simulink model "im_inv_sensorless_ctrl_model"  (R2026a)
settings: Solver=ode1  StopTime=simlength  FixedStep=tc  MaxStep=tc  EnableMultiTasking=on
values from neighbouring files (symbols this model uses):
  cp = 2    [im_param_calc_3.m]
  Ibez = Inom*sqrt(2)    [im_param_calc_3.m]
  Lm = Ls - Lds    [im_param_calc_3.m]
  Lr = Lm + Ldr    [im_param_calc_3.m]
  Ls = Vnom/sqrt(3)/I0/(2*pi*fnom)    [im_param_calc_3.m]
  Rr = Rr+deltaRr    (= 0.00099)    [im_param_calc_3.m]
  Rs = PhaseResistance    (= 0.009)    [im_param_calc_3.m]
undefined symbols (not defined in the file or in its folder): Adrso_im, alpha_norm, beta_norm, Crso_im, CTRPIFF_CLIP_RELEASE, dead_time, DiscIntNeverNeededParam, emf_fb_p, emf_p, fi_rot_ref_norm, fPWM_INV, gamma_norm, iq_lim, Jm_model, kg, ki_inv_d, ki_inv_q, ki_w, kp_inv_d, kp_inv_q, kp_w, kw, Ldrso_im, Lm_norm, Lr_norm, Ls_norm, magnitude, Omega_r_bez, Omega_s_bez, Rs_norm, sigma_norm, simlength, tc, Tcontrol_INV, timeRamp, Tload, ts_afe, ts_inv, uf_omega_ref, uf_uq_ref, wref
libraries: nesl_utility x64, fl_lib x49, simulink x2, im_uvw_2_lib x1, threephase_inductor_lib x1, cstblocks_lti x1
(part 1 of 4)
settings Model: SimulationMode=accelerator  Creator=LTNBDA  LastModifiedBy=ltnbda
settings SolverCC: ZeroCrossControl=EnableAll
settings DataIOCC: MaxDataPoints=1  SignalLoggingSaveFormat=ModelDataLogs
settings OptimizationCC: InitFltsAndDblsToZero=on
settings DebuggingCC: SaveWithParameterizedLinksMsg=none  UnderspecifiedInitializationDetection=Classic  SignalResolutionControl=TryResolveAllWithWarning  MultiTaskDSMMsg=warning  MultiTaskCondExecSysMsg=none  MultiTaskRateTransMsg=warning
settings HardwareCC: ProdBitPerLong=64.0  ProdHWDeviceType=Generic->64-bit Embedded Processor (LP64)
settings SFSimCC: SimCustomHeaderCode=|
  | #include "mavgflt.h"
  | #include "mavgflt_simulink.h"
  | #include "bemf_obsv.h"
  | #include "bemf_obsv_simulink.h"
  | #include "bemf_obsv_load_est.h"
  | #include "bemf_obsv_load_est_simulink.h"
  | #include "dqvector_pi.h"
  | #include "dqvector_pi_simulink.h"
  | #include "sv_pwm_simulink.h"
  | #include "sv_pwm.h"
settings SFSimCC: SimUserSources=|
  | "mavgflt_simulink.c"
  | "mavgflt.c"
  | "bemf_obsv_simulink.c"
  | "bemf_obsv.c"
  | "bemf_obsv_load_est_simulink.c"
  | "bemf_obsv_load_est.c"
  | "dqvector_pi.c"
  | "dqvector_pi_simulink.c"
  | "sv_pwm_simulink.c"
  | "sv_pwm.c"
settings SFSimCC: SimUserIncludeDirs=|
  | include
  | src
settings GRTTargetCC: TargetFcnLib=ansi_tfl_tmw.mat  CombineOutputUpdateFcns=off  GRTInterface=on
settings SimscapeCC: SimscapeNormalizeSystem=off  SimscapeNominalValues="[{\"value\":\"1\",\"unit\":\"A\"},{\"value\":\"1\",\"unit\":\"bar\"},{\"value\":\"1\",\"unit\":\"cm^2\"},{\"value\":\"1\",\"unit\":\"cm^3/s\"},{\"value\":\"1\",\"unit\":\"kJ/kg\"},{\"value\":\"1\",\"unit\":\"kW\"},{\"value\":\"1\",\"unit\":\"l\"},{\"value\":\"1\",\"unit\":\"N\"},{\"value\":\"1\",\"unit\":\"N*m\"},{\"value\":\"1\",\"unit\":\"V\"}]"  SimscapeLogType=none  SimscapeLogDataHistory=5000.0

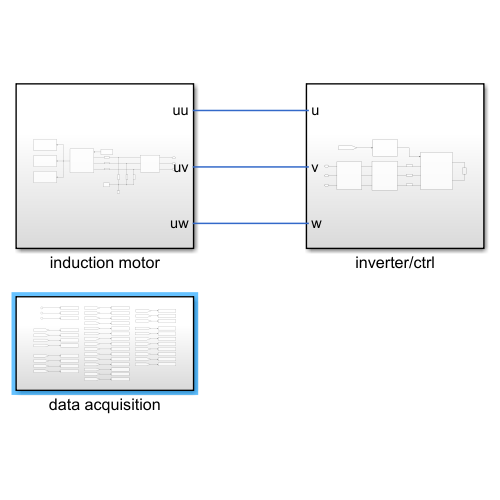
[thumbnail: Simulink's stored preview of the top-level diagram]
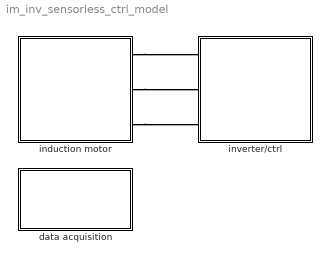
== system im_inv_sensorless_ctrl_model ==
  data acquisition : Subsystem
  induction motor : Subsystem
  inverter/ctrl : Subsystem
  connections:
  induction motor/RConn1 -- inverter/ctrl/LConn1
  induction motor/RConn2 -- inverter/ctrl/LConn2
  induction motor/RConn3 -- inverter/ctrl/LConn3

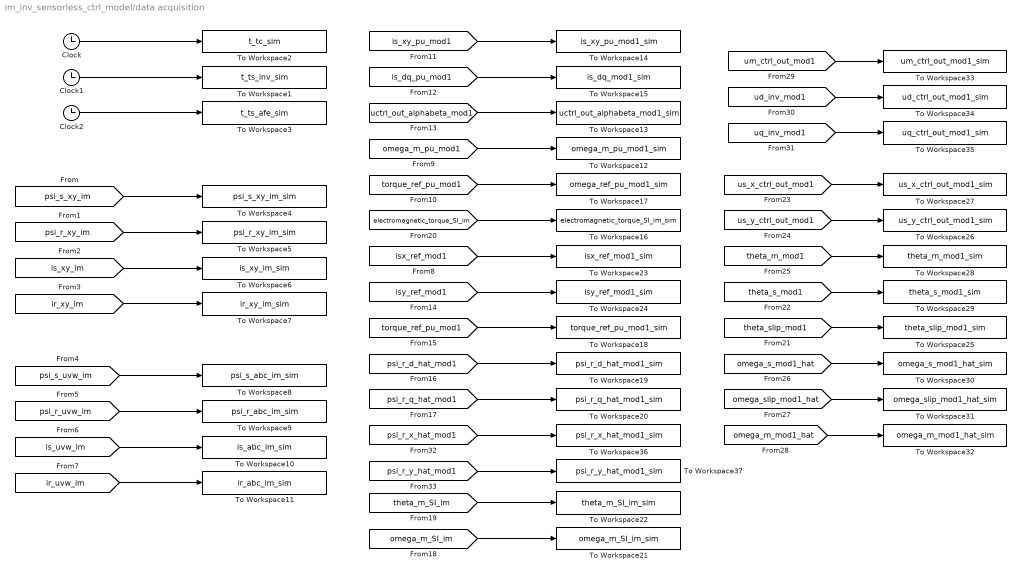
== system im_inv_sensorless_ctrl_model/data acquisition ==
  Clock : Clock
  Clock1 : Clock
  Clock2 : Clock
  To Workspace1 : ToWorkspace  VariableName=t_ts_inv_sim  SampleTime=ts_inv
      settings: MaxDataPoints=Ns_inv
  To Workspace10 : ToWorkspace  VariableName=is_abc_im_sim  SampleTime=tc
      settings: MaxDataPoints=Nc
  To Workspace11 : ToWorkspace  VariableName=ir_abc_im_sim  SampleTime=tc
      settings: MaxDataPoints=Nc
  To Workspace12 : ToWorkspace  VariableName=omega_m_pu_mod1_sim  SampleTime=ts_inv
      settings: MaxDataPoints=Ns_inv
  To Workspace13 : ToWorkspace  VariableName=uctrl_out_alphabeta_mod1_sim  SampleTime=ts_inv
      settings: MaxDataPoints=Ns_inv
  To Workspace14 : ToWorkspace  VariableName=is_xy_pu_mod1_sim  SampleTime=ts_inv
      settings: MaxDataPoints=Ns_inv
  To Workspace15 : ToWorkspace  VariableName=is_dq_mod1_sim  SampleTime=ts_inv
      settings: MaxDataPoints=Ns_inv
  To Workspace16 : ToWorkspace  VariableName=electromagnetic_torque_SI_im_sim  SampleTime=ts_inv
      settings: MaxDataPoints=Ns_inv
  To Workspace17 : ToWorkspace  VariableName=omega_ref_pu_mod1_sim  SampleTime=ts_inv
      settings: MaxDataPoints=Ns_inv
  To Workspace18 : ToWorkspace  VariableName=torque_ref_pu_mod1_sim  SampleTime=ts_inv
      settings: MaxDataPoints=Ns_inv
  To Workspace19 : ToWorkspace  VariableName=psi_r_d_hat_mod1_sim  SampleTime=ts_inv
      settings: MaxDataPoints=Ns_inv
  To Workspace2 : ToWorkspace  VariableName=t_tc_sim  SampleTime=tc
      settings: MaxDataPoints=Nc
  To Workspace20 : ToWorkspace  VariableName=psi_r_q_hat_mod1_sim  SampleTime=ts_inv
      settings: MaxDataPoints=Ns_inv
  To Workspace21 : ToWorkspace  VariableName=omega_m_SI_im_sim  SampleTime=ts_inv
      settings: MaxDataPoints=Ns_inv
  To Workspace22 : ToWorkspace  VariableName=theta_m_SI_im_sim  SampleTime=ts_inv
      settings: MaxDataPoints=Ns_inv
  To Workspace23 : ToWorkspace  VariableName=isx_ref_mod1_sim  SampleTime=ts_inv
      settings: MaxDataPoints=Ns_inv
  To Workspace24 : ToWorkspace  VariableName=isy_ref_mod1_sim  SampleTime=ts_inv
      settings: MaxDataPoints=Ns_inv
  To Workspace25 : ToWorkspace  VariableName=theta_slip_mod1_sim  SampleTime=ts_inv
      settings: MaxDataPoints=Ns_inv
  To Workspace26 : ToWorkspace  VariableName=us_y_ctrl_out_mod1_sim  SampleTime=ts_inv
      settings: MaxDataPoints=Ns_afe
  To Workspace27 : ToWorkspace  VariableName=us_x_ctrl_out_mod1_sim  SampleTime=ts_inv
      settings: MaxDataPoints=Ns_afe
  To Workspace28 : ToWorkspace  VariableName=theta_m_mod1_sim  SampleTime=ts_inv
      settings: MaxDataPoints=Ns_inv
  To Workspace29 : ToWorkspace  VariableName=theta_s_mod1_sim  SampleTime=ts_inv
      settings: MaxDataPoints=Ns_inv
  To Workspace3 : ToWorkspace  VariableName=t_ts_afe_sim  SampleTime=ts_afe
      settings: MaxDataPoints=Ns_afe
  To Workspace30 : ToWorkspace  VariableName=omega_s_mod1_hat_sim  SampleTime=ts_inv
      settings: MaxDataPoints=Ns_inv
  To Workspace31 : ToWorkspace  VariableName=omega_slip_mod1_hat_sim  SampleTime=ts_inv
      settings: MaxDataPoints=Ns_inv
  To Workspace32 : ToWorkspace  VariableName=omega_m_mod1_hat_sim  SampleTime=ts_inv
      settings: MaxDataPoints=Ns_inv
  To Workspace33 : ToWorkspace  VariableName=um_ctrl_out_mod1_sim  SampleTime=ts_inv
      settings: MaxDataPoints=Ns_afe
  To Workspace34 : ToWorkspace  VariableName=ud_ctrl_out_mod1_sim  SampleTime=ts_inv
      settings: MaxDataPoints=Ns_afe
  To Workspace35 : ToWorkspace  VariableName=uq_ctrl_out_mod1_sim  SampleTime=ts_inv
      settings: MaxDataPoints=Ns_afe
  To Workspace36 : ToWorkspace  VariableName=psi_r_x_hat_mod1_sim  SampleTime=ts_inv
      settings: MaxDataPoints=Ns_inv
  To Workspace37 : ToWorkspace  VariableName=psi_r_y_hat_mod1_sim  SampleTime=ts_inv
      settings: MaxDataPoints=Ns_inv
  To Workspace4 : ToWorkspace  VariableName=psi_s_xy_im_sim  SampleTime=tc
      settings: MaxDataPoints=Nc
  To Workspace5 : ToWorkspace  VariableName=psi_r_xy_im_sim  SampleTime=tc
      settings: MaxDataPoints=Nc
  To Workspace6 : ToWorkspace  VariableName=is_xy_im_sim  SampleTime=tc
      settings: MaxDataPoints=Nc
  To Workspace7 : ToWorkspace  VariableName=ir_xy_im_sim  SampleTime=tc
      settings: MaxDataPoints=Nc
  To Workspace8 : ToWorkspace  VariableName=psi_s_abc_im_sim  SampleTime=tc
      settings: MaxDataPoints=Nc
  To Workspace9 : ToWorkspace  VariableName=psi_r_abc_im_sim  SampleTime=tc
      settings: MaxDataPoints=Nc
  wires:
  Clock/1 -> To Workspace2/1
  Clock1/1 -> To Workspace1/1
  Clock2/1 -> To Workspace3/1
  [psi_s_xy_im] -> To Workspace4/1
  [psi_r_xy_im] -> To Workspace5/1
  [is_xy_im] -> To Workspace6/1
  [ir_xy_im] -> To Workspace7/1
  [psi_s_uvw_im] -> To Workspace8/1
  [psi_r_uvw_im] -> To Workspace9/1
  [is_uvw_im] -> To Workspace10/1
  [ir_uvw_im] -> To Workspace11/1
  [is_dq_pu_mod1] -> To Workspace15/1
  [uctrl_out_alphabeta_mod1] -> To Workspace13/1
  [is_xy_pu_mod1] -> To Workspace14/1
  [omega_m_pu_mod1] -> To Workspace12/1
  [electromagnetic_torque_SI_im] -> To Workspace16/1
  [torque_ref_pu_mod1] -> To Workspace17/1
  [omega_m_SI_im] -> To Workspace21/1
  [torque_ref_pu_mod1] -> To Workspace18/1
  [psi_r_d_hat_mod1] -> To Workspace19/1
  [psi_r_q_hat_mod1] -> To Workspace20/1
  [theta_m_SI_im] -> To Workspace22/1
  [isx_ref_mod1] -> To Workspace23/1
  [isy_ref_mod1] -> To Workspace24/1
  [theta_slip_mod1] -> To Workspace25/1
  [us_x_ctrl_out_mod1] -> To Workspace27/1
  [us_y_ctrl_out_mod1] -> To Workspace26/1
  [theta_m_mod1] -> To Workspace28/1
  [theta_s_mod1] -> To Workspace29/1
  [omega_s_mod1_hat] -> To Workspace30/1
  [omega_slip_mod1_hat] -> To Workspace31/1
  [omega_m_mod1_hat] -> To Workspace32/1
  [um_ctrl_out_mod1] -> To Workspace33/1
  [ud_inv_mod1] -> To Workspace34/1
  [uq_inv_mod1] -> To Workspace35/1
  [psi_r_x_hat_mod1] -> To Workspace36/1
  [psi_r_y_hat_mod1] -> To Workspace37/1

== system im_inv_sensorless_ctrl_model/induction motor ==
  Electrical Reference : fl_lib/Electrical/Electrical Elements/Electrical Reference
  Inductor : fl_lib/Electrical/Electrical Elements/Inductor  l=1e-6 H  r=0 Ohm  g=1e-9 1/Ohm  i_specify=off  i_priority=None  i=0 A  i_nominal_specify=off  i_nominal_value=1  i_nominal_unit=A  v_specify=off  v_priority=None  v=0 V  v_nominal_specify=off  v_nominal_value=1  v_nominal_unit=V  i_L_specify=off  i_L_priority=High  i_L=0 A  i_L_nominal_specify=off  i_L_nominal_value=1  i_L_nominal_unit=A
  Inductor1 : fl_lib/Electrical/Electrical Elements/Inductor  l=1e-6 H  r=0 Ohm  g=1e-9 1/Ohm  i_specify=off  i_priority=None  i=0 A  i_nominal_specify=off  i_nominal_value=1  i_nominal_unit=A  v_specify=off  v_priority=None  v=0 V  v_nominal_specify=off  v_nominal_value=1  v_nominal_unit=V  i_L_specify=off  i_L_priority=High  i_L=0 A  i_L_nominal_specify=off  i_L_nominal_value=1  i_L_nominal_unit=A
  Inductor2 : fl_lib/Electrical/Electrical Elements/Inductor  l=1e-6 H  r=0 Ohm  g=1e-9 1/Ohm  i_specify=off  i_priority=None  i=0 A  i_nominal_specify=off  i_nominal_value=1  i_nominal_unit=A  v_specify=off  v_priority=None  v=0 V  v_nominal_specify=off  v_nominal_value=1  v_nominal_unit=V  i_L_specify=off  i_L_priority=High  i_L=0 A  i_L_nominal_specify=off  i_L_nominal_value=1  i_L_nominal_unit=A
  Resistor : fl_lib/Electrical/Electrical Elements/Resistor  R=1e5 Ohm  i_specify=off  i_priority=None  i=0 A  i_nominal_specify=off  i_nominal_value=1  i_nominal_unit=A  v_specify=off  v_priority=None  v=0 V  v_nominal_specify=off  v_nominal_value=1  v_nominal_unit=V
  Resistor1 : fl_lib/Electrical/Electrical Elements/Resistor  R=1e5 Ohm  i_specify=off  i_priority=None  i=0 A  i_nominal_specify=off  i_nominal_value=1  i_nominal_unit=A  v_specify=off  v_priority=None  v=0 V  v_nominal_specify=off  v_nominal_value=1  v_nominal_unit=V
  Resistor2 : fl_lib/Electrical/Electrical Elements/Resistor  R=1e5 Ohm  i_specify=off  i_priority=None  i=0 A  i_nominal_specify=off  i_nominal_value=1  i_nominal_unit=A  v_specify=off  v_priority=None  v=0 V  v_nominal_specify=off  v_nominal_value=1  v_nominal_unit=V
  Solver Configuration : nesl_utility/Solver Configuration  PhysicalDomain=network_engine_domain  SubClassName=solver  LeftPortType=input  RightPortType=generic  Tones=[]  Harmonics=[]  SimulateNoise=off  Profile=off  UseLocalSampling=off  EnableSwitchedLinearOptims=on  FrequencyDomain=off  UseCCode=off  RelTol=0.001  AbsTol=0.001  MinStep=1e-09  ToWorkspace=off  RevertToSquareIcSolve=off  NumHomotopyIterations=100  PhasorMode=off  PhasorModeNumHarmonics=1  ConsistencySolver=NEWTON_XTOL_AFTER_FTOL  CanonicalOrdering=UNORDERED  OptimizeIntermediates=UNOPTIMIZED  IndexReductionMethod=DerivativeReplacement  DoDC=off  ResidualTolerance=1e-09  ConsistencyTolSource=GLOBAL  ConsistencyAbsTol=0.001  ConsistencyRelTol=0.001  ConsistencyTolFactor=0.001  UseLocalSolver=on  LocalSolverChoice=NE_BACKWARD_EULER_ADVANCER  ResolveIndetEquations=on  FunctionEvalNumThread=1  LocalSolverSampleTime=tc  DoFixedCost=on  MaxNonlinIter=3  MaxModeIter=2  ComputeImpulses=off  ImpulseIterations=2  LinearAlgebra=auto  LinearAlgebraNumThread=0  EquationFormulation=NE_TIME_EF  DelaysMemoryBudget=1024  AutomaticFiltering=on  FilteringTimeConstant=0.001  PartitionStorageMethod=AS_NEEDED  PartitionMemoryBudget=1024  PartitionMethod=ROBUST  MultibodyUseLocalSolver=off  MultibodyLocalSolverChoice=ODE1  MultibodyLocalSolverSampleTime=0.001
  control performance evaluation : Subsystem
  induction motor : Subsystem
  load generator : Subsystem
  machine performance evaluation : Subsystem
  mechanical data : Subsystem
  threephase_vi_measures_stack : Subsystem
  uu : PMIOPort  Side=Right
  uv : PMIOPort  Port=2  Side=Right
  uw : PMIOPort  Port=3  Side=Right
  wires:
  induction motor/1(motor_data) -> control performance evaluation/1(machine_data), machine performance evaluation/1(machine_data), mechanical data/1(machine data)
  load generator/1(torque) -> induction motor/1(torque load)
  connections:
  induction motor/LConn2 -- Inductor1/LConn1
  Resistor/LConn1 -- threephase_vi_measures_stack/RConn1 -- Inductor/RConn1
  induction motor/LConn3 -- Inductor2/LConn1
  induction motor/LConn1 -- Inductor/LConn1
  Resistor1/LConn1 -- threephase_vi_measures_stack/RConn2 -- Inductor1/RConn1
  Resistor2/LConn1 -- threephase_vi_measures_stack/RConn3 -- Inductor2/RConn1
  Resistor/RConn1 -- Solver Configuration/RConn1 -- Resistor2/RConn1 -- Resistor1/RConn1 -- Electrical Reference/LConn1
  threephase_vi_measures_stack/LConn1 -- uu/RConn1
  threephase_vi_measures_stack/LConn2 -- uv/RConn1
  threephase_vi_measures_stack/LConn3 -- uw/RConn1

== system im_inv_sensorless_ctrl_model/inverter//ctrl ==
  DC Voltage Source : fl_lib/Electrical/Electrical Sources/DC Voltage Source  v0=Vdc_ref V
  Inductor : fl_lib/Electrical/Electrical Elements/Inductor  l=1e-6 H  r=0 Ohm  g=1e-9 1/Ohm  i_specify=off  i_priority=None  i=0 A  i_nominal_specify=off  i_nominal_value=1  i_nominal_unit=A  v_specify=off  v_priority=None  v=0 V  v_nominal_specify=off  v_nominal_value=1  v_nominal_unit=V  i_L_specify=off  i_L_priority=High  i_L=0 A  i_L_nominal_specify=off  i_L_nominal_value=1  i_L_nominal_unit=A
  Inductor1 : fl_lib/Electrical/Electrical Elements/Inductor  l=1e-6 H  r=0 Ohm  g=1e-9 1/Ohm  i_specify=off  i_priority=None  i=0 A  i_nominal_specify=off  i_nominal_value=1  i_nominal_unit=A  v_specify=off  v_priority=None  v=0 V  v_nominal_specify=off  v_nominal_value=1  v_nominal_unit=V  i_L_specify=off  i_L_priority=High  i_L=0 A  i_L_nominal_specify=off  i_L_nominal_value=1  i_L_nominal_unit=A
  Inductor2 : fl_lib/Electrical/Electrical Elements/Inductor  l=1e-6 H  r=0 Ohm  g=1e-9 1/Ohm  i_specify=off  i_priority=None  i=0 A  i_nominal_specify=off  i_nominal_value=1  i_nominal_unit=A  v_specify=off  v_priority=None  v=0 V  v_nominal_specify=off  v_nominal_value=1  v_nominal_unit=V  i_L_specify=off  i_L_priority=High  i_L=0 A  i_L_nominal_specify=off  i_L_nominal_value=1  i_L_nominal_unit=A
  LFi : threephase_inductor_lib/threephase inductor  Lp=LFi_d H  L0=LFi_0 H  Rp=RLFi_d Ohm  R0=RLFi_0 Ohm  Lls=5e-6 H  uu_1_specify=off  uu_1_priority=None  uu_1=0 V  uu_1_nominal_specify=off  uu_1_nominal_value=1  uu_1_nominal_unit=V  uv_1_specify=off  uv_1_priority=None  uv_1=0 V  uv_1_nominal_specify=off  uv_1_nominal_value=1  uv_1_nominal_unit=V  uw_1_specify=off  uw_1_priority=None  uw_1=0 V  uw_1_nominal_specify=off  uw_1_nominal_value=1  uw_1_nominal_unit=V  uu_2_specify=off  uu_2_priority=None  uu_2=0 V  uu_2_nominal_specify=off  uu_2_nominal_value=1  uu_2_nominal_unit=V  uv_2_specify=off  uv_2_priority=None  uv_2=0 V  uv_2_nominal_specify=off  uv_2_nominal_value=1  uv_2_nominal_unit=V  uw_2_specify=off  uw_2_priority=None  uw_2=0 V  uw_2_nominal_specify=off  uw_2_nominal_value=1  uw_2_nominal_unit=V  iu_specify=off  iu_priority=None  iu=0 A  iu_nominal_specify=off  iu_nominal_value=1  iu_nominal_unit=A  iv_specify=off  iv_priority=None  iv=0 A  iv_nominal_specify=off  iv_nominal_value=1  iv_nominal_unit=A  iw_specify=off  iw_priority=None  iw=0 A  iw_nominal_specify=off  iw_nominal_value=1  iw_nominal_unit=A
  im_ctrl : Subsystem
  inverter : Subsystem
  threephase_vi_measures_stack : Subsystem
  u : PMIOPort  Side=Left
  v : PMIOPort  Port=2  Side=Left
  w : PMIOPort  Port=3  Side=Left
  wires:
  [theta_m_mod1] -> im_ctrl/1(theta_m)
  im_ctrl/1(u_ctrl_alphabeta) -> inverter/1(uab)
  connections:
  LFi/RConn1 -- Inductor/LConn1
  Inductor1/LConn1 -- LFi/RConn2
  LFi/RConn3 -- Inductor2/LConn1
  threephase_vi_measures_stack/LConn1 -- LFi/LConn1
  threephase_vi_measures_stack/LConn2 -- LFi/LConn2
  threephase_vi_measures_stack/LConn3 -- LFi/LConn3
  threephase_vi_measures_stack/RConn3 -- w/RConn1
  threephase_vi_measures_stack/RConn2 -- v/RConn1
  threephase_vi_measures_stack/RConn1 -- u/RConn1
  inverter/LConn1 -- Inductor/RConn1
  inverter/LConn2 -- Inductor1/RConn1
  inverter/LConn3 -- Inductor2/RConn1
  DC Voltage Source/LConn1 -- inverter/RConn1
  DC Voltage Source/RConn1 -- inverter/RConn2

== system im_inv_sensorless_ctrl_model/induction motor/control performance evaluation ==
  machine_data : Inport
  adc2dq_s_1 : Subsystem
  adc2dq_s_2 : Subsystem
  adc2dq_slip_1 : Subsystem
  adc2dq_slip_2 : Subsystem
  ir_uvw : BusSelector  OutputSignals=iru(A),irv(A),irw(A)  OutputAsBus=on
  is_uvw : BusSelector  OutputSignals=isu(A),isv(A),isw(A)  OutputAsBus=on
  psi_r_uvw : BusSelector  OutputSignals=psi_r_u(Vs),psi_r_v(Vs),psi_r_w(Vs)  OutputAsBus=on
  psi_s_uvw : BusSelector  OutputSignals=psi_s_u(Vs),psi_s_v(Vs),psi_s_w(Vs)  OutputAsBus=on
  stator/rotor uvw currents : Scope  NumInputPorts=2
      settings: ActiveDisplayYMinimum=-569.7187250347755  ActiveDisplayYMaximum=580.7473381124961  DataLoggingVariableName=ScopeData15
  stator/rotor uvw fluxes : Scope  NumInputPorts=2
      settings: ActiveDisplayYMinimum=-1.236467692960036  ActiveDisplayYMaximum=1.3517472693614645  DataLoggingVariableName=ScopeData16
  stator/rotor xy currents : Scope  NumInputPorts=2
      settings: ActiveDisplayYMinimum=-2297.8110392737149  ActiveDisplayYMaximum=257.87338844640192
  stator/rotor xy fluxes : Scope  NumInputPorts=2
      settings: ActiveDisplayYMinimum=-2.073456127351001  ActiveDisplayYMaximum=0.70751576648044434  DataLoggingVariableName=ScopeData2
  tag scope: ir_uvw_im=global, is_uvw_im=global, psi_r_uvw_im=global, psi_s_uvw_im=global
  wires:
  machine_data/1 -> psi_s_uvw/1, psi_r_uvw/1, is_uvw/1, ir_uvw/1
  psi_s_uvw/1 -> [psi_s_uvw_im], adc2dq_s_1/1(abc)
  adc2dq_s_1/1(dq) -> stator/rotor xy fluxes/1  "psi_s_xy"
  psi_r_uvw/1 -> [psi_r_uvw_im], adc2dq_slip_1/1(abc)
  adc2dq_slip_1/1(dq) -> stator/rotor xy fluxes/2  "psi_r_xy"
  adc2dq_slip_2/1(dq) -> stator/rotor xy currents/2  "ir_xy"
  adc2dq_s_2/1(dq) -> stator/rotor xy currents/1  "is_xy"
  is_uvw/1 -> [is_uvw_im], adc2dq_s_2/1(abc)
  ir_uvw/1 -> [ir_uvw_im], adc2dq_slip_2/1(abc)
  [is_uvw_im] -> stator/rotor uvw currents/1
  [ir_uvw_im] -> stator/rotor uvw currents/2
  [psi_r_uvw_im] -> stator/rotor uvw fluxes/2
  [psi_s_uvw_im] -> stator/rotor uvw fluxes/1

== system im_inv_sensorless_ctrl_model/induction motor/induction motor ==
  torque load : Inport
  Gain : Gain  Gain=-1
  Ideal Rotational Motion Sensor : fl_lib/Mechanical/Mechanical Sensors/Ideal Rotational Motion Sensor  reference=foundation.enum.MeasurementReference.difference  acceleration_port=false  velocity_port=true  position_port=true  wrap_angle=false  offset=0 rad
  Ideal Torque Source : fl_lib/Mechanical/Mechanical Sources/Ideal Torque Source
  Mechanical Rotational Reference : fl_lib/Mechanical/Rotational Elements/Mechanical Rotational Reference
  Mechanical Rotational Reference1 : fl_lib/Mechanical/Rotational Elements/Mechanical Rotational Reference
  Open Circuit : fl_lib/Electrical/Electrical Elements/Open Circuit  v_specify=off  v_priority=None  v=0 V  v_nominal_specify=off  v_nominal_value=1  v_nominal_unit=V
  PS Gain : fl_lib/Physical Signals/Functions/PS Gain  gain=-1
  PS Transfer Function : fl_lib/Physical Signals/Linear Operators/PS Transfer Function  transfer_function_type=foundation.enum.transfer_function_type.lag  T=1/50 s  T1=2 s  T2=1 s  reset_method=foundation.enum.IntegratorResetSpec.None  initial_condition_spec=foundation.enum.IntegratorICSpec.Internal  y0=0 N*m
  PS-Simulink Converter24 : nesl_utility/PS-Simulink Converter  PhysicalDomain=network_engine_domain  SubClassName=ps_output  LeftPortType=input  RightPortType=output  PseudoPeriodic=off  Frequencies=[]  VectorFormat=1-D array  Unit=rad  AffineConversion=off
  Simulink-PS Converter : nesl_utility/Simulink-PS Converter  PhysicalDomain=network_engine_domain  SubClassName=ps_input  LeftPortType=input  RightPortType=output  PseudoPeriodic=off  Frequencies=[]  NoiseDistribution=none  NoiseParameters=[]  Unit=N*m  AffineConversion=off  FilteringAndDerivatives=provide  SimscapeFilterOrder=1  InputFilterTimeConstant=0.001  UdotUserProvided=0
  im : Subsystem  mask{Rs=Rs, Ls=Ls, Lm=Lm, Lr=Lr, Rr=Rr, Jm=Jm_model, bm=Tn/omega_m_nom/3, pp=cp}
      mask prompts: Rs "Stator resistance - Rs(Ohm)"; Ls "Stator inductance - Ls(H)"; Lm "Mutual inductance - Ls(H)"; Lr "Rotor inductance - Ls(H)"; Rr "Rotor resistance - Rs(Ohm)"; Jm "Total moment of inertia - Jm (kgm^2)"; bm "Rotational viscosity - bm (Nm*s/rad)"; pp "Number of pole pairs"
      mask Display:
      | disp('IM');
      | port_label('lconn', 1, 'u');
      | port_label('lconn', 2, 'v');
      | port_label('lconn', 3, 'w');
      | port_label('lconn', 4, 'n');
      | port_label('output', 1, 'motor data');
      | port_label('rconn',1, 'S');
  uu : PMIOPort  Side=Left
  uv : PMIOPort  Port=2  Side=Left
  uw : PMIOPort  Port=3  Side=Left
  motor_data : Outport
  tag scope: rotor_phase_m_encoder=global
  wires:
  torque load/1 -> Simulink-PS Converter/1
  PS-Simulink Converter24/1 -> Gain/1
  Gain/1 -> [rotor_phase_m_encoder]
  im/1(motor_data) -> motor_data/1
  connections:
  Ideal Torque Source/LConn1 -- im/RConn1 -- Ideal Rotational Motion Sensor/RConn1
  Mechanical Rotational Reference/LConn1 -- Ideal Torque Source/RConn2
  PS Transfer Function/RConn1 -- PS Gain/LConn1
  Simulink-PS Converter/RConn1 -- PS Transfer Function/LConn1
  PS Gain/RConn1 -- Ideal Torque Source/RConn1
  Mechanical Rotational Reference1/LConn1 -- Ideal Rotational Motion Sensor/LConn1
  Ideal Rotational Motion Sensor/RConn3 -- PS-Simulink Converter24/LConn1
  im/LConn1 -- uu/RConn1
  im/LConn2 -- uv/RConn1
  im/LConn3 -- uw/RConn1
  Open Circuit/LConn1 -- im/LConn4

== system im_inv_sensorless_ctrl_model/induction motor/load generator ==
  Gain3 : Gain
  RampSlow : simulink/Sources/Ramp  slope=Tload/timeRamp/simlength*2  start=start_load_ramp  InitialOutput=0
  Saturation : Saturate  UpperLimit=Tload  LowerLimit=-Tload
  Step : Step  FinalValue=Tload  SampleTime=0
  torque : Outport
  wires:
  Gain3/1 -> torque/1
  RampSlow/1 -> Saturation/1
  Step/1 -> Gain3/1

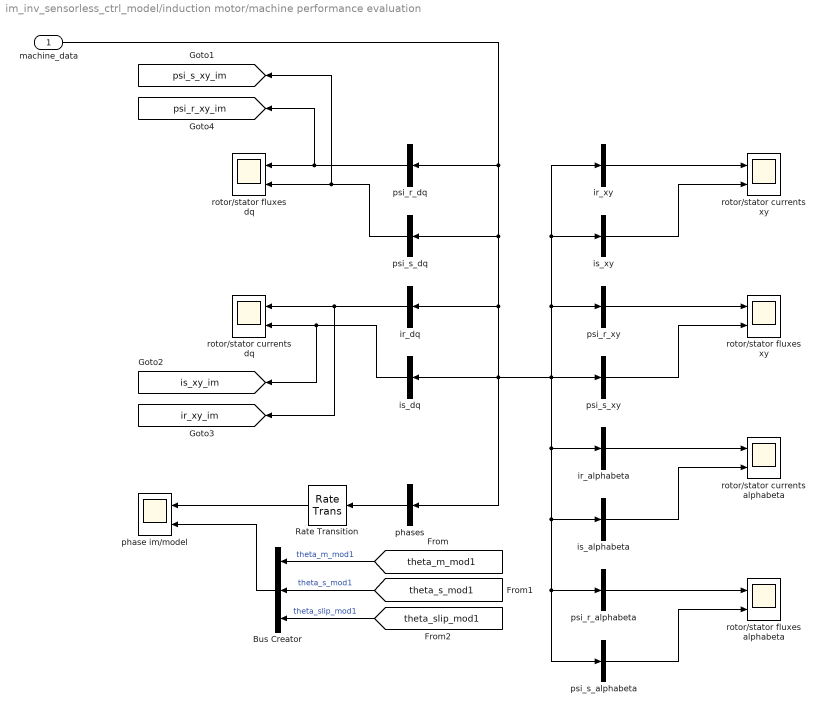
== system im_inv_sensorless_ctrl_model/induction motor/machine performance evaluation ==
  machine_data : Inport
  Bus Creator : BusCreator  Inputs=3
  Rate Transition : RateTransition
  ir_alphabeta : BusSelector  OutputSignals=ir_alpha(A),ir_beta(A)  OutputAsBus=on
  ir_dq : BusSelector  OutputSignals=ird(A),irq(A)  OutputAsBus=on
  ir_xy : BusSelector  OutputSignals=irx(A),iry(A)  OutputAsBus=on
  is_alphabeta : BusSelector  OutputSignals=is_alpha(A),is_beta(A)  OutputAsBus=on
  is_dq : BusSelector  OutputSignals="isd  (A),isq(A)"  OutputAsBus=on
  is_xy : BusSelector  OutputSignals=isx(A),isy(A)  OutputAsBus=on
  phase im/model : Scope  NumInputPorts=2
      settings: ActiveDisplayYMinimum=-3.9265862737533843  ActiveDisplayYMaximum=3.9260094563988228  DataLoggingVariableName=ScopeData17
  phases : BusSelector  OutputSignals=rotor_phase_electrical(rad),stator_phase_electrical(rad),slip_phase_electrical(rad)  OutputAsBus=on
  psi_r_alphabeta : BusSelector  OutputSignals=psi_r_alpha(Vs),psi_r_beta(Vs)  OutputAsBus=on
  psi_r_dq : BusSelector  OutputSignals=psi_r_d(Vs),psi_r_q(Vs)  OutputAsBus=on
  psi_r_xy : BusSelector  OutputSignals=psi_r_x(Vs),psi_r_y(Vs)  OutputAsBus=on
  psi_s_alphabeta : BusSelector  OutputSignals=psi_s_alpha(Vs),psi_s_beta(Vs)  OutputAsBus=on
  psi_s_dq : BusSelector  OutputSignals=psi_s_d(Vs),psi_s_q(Vs)  OutputAsBus=on
  psi_s_xy : BusSelector  OutputSignals=psi_s_x(Vs),psi_s_y(Vs)  OutputAsBus=on
  rotor/stator currents alphabeta : Scope  NumInputPorts=2
      settings: ActiveDisplayYMinimum=-755.39541757603456  ActiveDisplayYMaximum=755.78854721223524  DataLoggingVariableName=ScopeData13
  rotor/stator currents dq : Scope  NumInputPorts=2
      settings: ActiveDisplayYMinimum=-890.18338057152221  ActiveDisplayYMaximum=1029.0815378849704  DataLoggingVariableName=ScopeData3
  rotor/stator currents xy : Scope  NumInputPorts=2
      settings: ActiveDisplayYMinimum=-752.721270314659  ActiveDisplayYMaximum=755.87183047398014  DataLoggingVariableName=ScopeData6
  rotor/stator fluxes alphabeta : Scope  NumInputPorts=2
      settings: ActiveDisplayYMinimum=-2.3042822009960924  ActiveDisplayYMaximum=2.3048133761652672  DataLoggingVariableName=ScopeData14
  rotor/stator fluxes dq : Scope  NumInputPorts=2
      settings: ActiveDisplayYMinimum=-1.3704704510731207  ActiveDisplayYMaximum=1.3704905297766097
  rotor/stator fluxes xy : Scope  NumInputPorts=2
      settings: ActiveDisplayYMinimum=-2.5178704524257092  ActiveDisplayYMaximum=0.44165401935710158  DataLoggingVariableName=ScopeData12
  tag scope: ir_xy_im=global, is_xy_im=global, psi_r_xy_im=global, psi_s_xy_im=global
  wires:
  psi_r_dq/1 -> [psi_r_xy_im], rotor/stator fluxes dq/1
  psi_s_dq/1 -> [psi_s_xy_im], rotor/stator fluxes dq/2
  ir_dq/1 -> [ir_xy_im], rotor/stator currents dq/1
  is_dq/1 -> [is_xy_im], rotor/stator currents dq/2
  is_xy/1 -> rotor/stator currents xy/2
  ir_xy/1 -> rotor/stator currents xy/1
  psi_r_xy/1 -> rotor/stator fluxes xy/1
  psi_s_xy/1 -> rotor/stator fluxes xy/2
  psi_s_alphabeta/1 -> rotor/stator fluxes alphabeta/2
  psi_r_alphabeta/1 -> rotor/stator fluxes alphabeta/1
  machine_data/1 -> psi_r_dq/1, ir_dq/1, phases/1, psi_s_alphabeta/1, psi_r_alphabeta/1, is_alphabeta/1, ir_alphabeta/1, psi_s_xy/1, ir_xy/1, is_xy/1, psi_r_xy/1, is_dq/1, psi_s_dq/1
  ir_alphabeta/1 -> rotor/stator currents alphabeta/1
  is_alphabeta/1 -> rotor/stator currents alphabeta/2
  phases/1 -> Rate Transition/1
  [theta_m_mod1] -> Bus Creator/1  "theta_m_mod1"
  [theta_slip_mod1] -> Bus Creator/3  "theta_slip_mod1"
  Bus Creator/1 -> phase im/model/2
  [theta_s_mod1] -> Bus Creator/2  "theta_s_mod1"
  Rate Transition/1 -> phase im/model/1

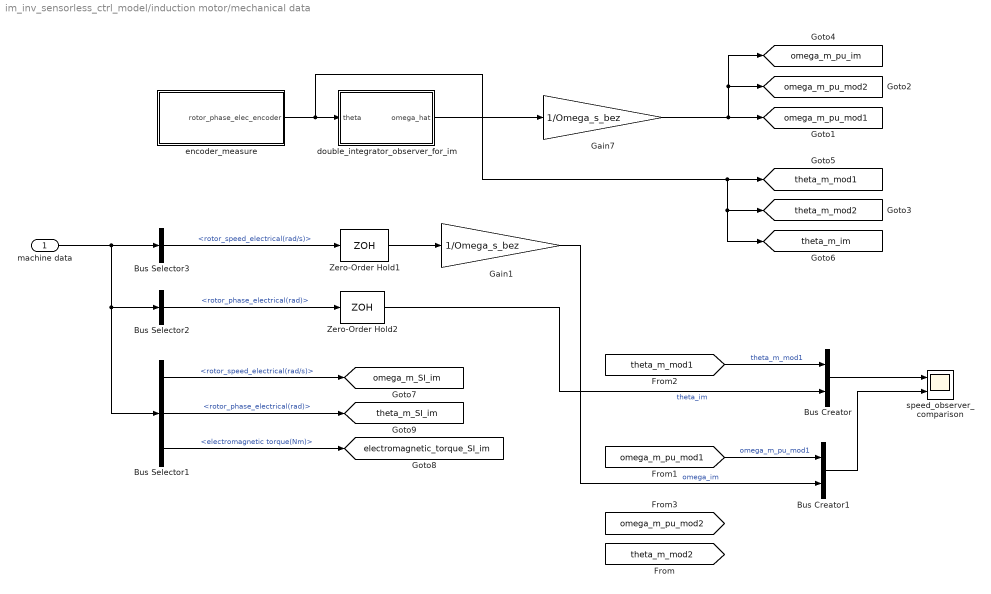
== system im_inv_sensorless_ctrl_model/induction motor/mechanical data ==
  machine data : Inport
  Bus Creator : BusCreator  Inputs=2
  Bus Creator1 : BusCreator  Inputs=2
  Bus Selector1 : BusSelector  OutputSignals=rotor_speed_electrical(rad/s),rotor_phase_electrical(rad),electromagnetic torque(Nm)
  Bus Selector2 : BusSelector  OutputSignals=rotor_phase_electrical(rad)
  Bus Selector3 : BusSelector  OutputSignals=rotor_speed_electrical(rad/s)
  Gain1 : Gain  Gain=1/Omega_s_bez
  Gain7 : Gain  Gain=1/Omega_s_bez
  Zero-Order Hold1 : ZeroOrderHold  SampleTime=ts_inv
  Zero-Order Hold2 : ZeroOrderHold  SampleTime=ts_inv
  double_integrator_observer_for_im : Subsystem
  encoder_measure : Subsystem
  speed_observer_comparison : Scope  NumInputPorts=2
      settings: ActiveDisplayYMinimum=-1.1236576045068563  ActiveDisplayYMaximum=1.1217366799891755  DataLoggingVariableName=ScopeData8
  tag scope: electromagnetic_torque_SI_im=global, omega_m_SI_im=global, omega_m_pu_im=global, omega_m_pu_mod1=global, omega_m_pu_mod2=global, theta_m_SI_im=global, theta_m_im=global, theta_m_mod1=global, theta_m_mod2=global
  wires:
  encoder_measure/1(rotor_phase_elec_encoder) -> [theta_m_mod1], [theta_m_im], [theta_m_mod2], double_integrator_observer_for_im/1(theta)
  machine data/1 -> Bus Selector1/1, Bus Selector2/1, Bus Selector3/1
  Bus Selector3/1 -> Zero-Order Hold1/1  "<rotor_speed_electrical(rad/s)>"
  Bus Selector2/1 -> Zero-Order Hold2/1  "<rotor_phase_electrical(rad)>"
  Gain7/1 -> [omega_m_pu_mod1], [omega_m_pu_mod2], [omega_m_pu_im]
  Bus Selector1/1 -> [omega_m_SI_im]  "<rotor_speed_electrical(rad/s)>"
  Bus Selector1/3 -> [electromagnetic_torque_SI_im]  "<electromagnetic torque(Nm)>"
  Bus Selector1/2 -> [theta_m_SI_im]  "<rotor_phase_electrical(rad)>"
  double_integrator_observer_for_im/1(omega_hat) -> Gain7/1
  [theta_m_mod1] -> Bus Creator/1  "theta_m_mod1"
  [omega_m_pu_mod1] -> Bus Creator1/1  "omega_m_pu_mod1"
  Bus Creator/1 -> speed_observer_comparison/1
  Bus Creator1/1 -> speed_observer_comparison/2
  Zero-Order Hold2/1 -> Bus Creator/2  "theta_im"
  Zero-Order Hold1/1 -> Gain1/1
  Gain1/1 -> Bus Creator1/2  "omega_im"

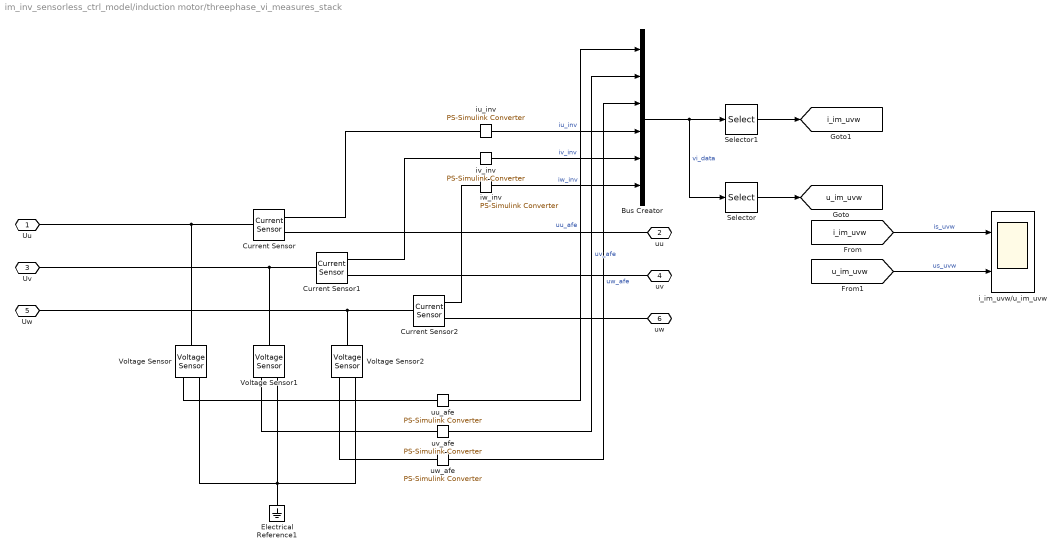
== system im_inv_sensorless_ctrl_model/induction motor/threephase_vi_measures_stack ==
  Bus Creator : BusCreator  Inputs=6
  Current Sensor : fl_lib/Electrical/Electrical Sensors/Current Sensor
  Current Sensor1 : fl_lib/Electrical/Electrical Sensors/Current Sensor
  Current Sensor2 : fl_lib/Electrical/Electrical Sensors/Current Sensor
  Electrical Reference1 : fl_lib/Electrical/Electrical Elements/Electrical Reference
  Selector : Selector  InputPortWidth=6  IndexOptions=Index vector (dialog)  Indices=[1 2 3]  OutputSizes=1
  Selector1 : Selector  InputPortWidth=6  IndexOptions=Index vector (dialog)  Indices=[4 5 6]  OutputSizes=1
  Voltage Sensor : fl_lib/Electrical/Electrical Sensors/Voltage Sensor
  Voltage Sensor1 : fl_lib/Electrical/Electrical Sensors/Voltage Sensor
  Voltage Sensor2 : fl_lib/Electrical/Electrical Sensors/Voltage Sensor
  i_im_uvw/u_im_uvw : Scope  NumInputPorts=2
      settings: SampleTime=tc  ActiveDisplayYMinimum=-552.59990522028443  ActiveDisplayYMaximum=552.59841185091216
  iu_inv : nesl_utility/PS-Simulink Converter  PhysicalDomain=network_engine_domain  SubClassName=ps_output  LeftPortType=input  RightPortType=output  PseudoPeriodic=off  Frequencies=[]  VectorFormat=1-D array  Unit=A  AffineConversion=off
  iv_inv : nesl_utility/PS-Simulink Converter  PhysicalDomain=network_engine_domain  SubClassName=ps_output  LeftPortType=input  RightPortType=output  PseudoPeriodic=off  Frequencies=[]  VectorFormat=1-D array  Unit=A  AffineConversion=off
  iw_inv : nesl_utility/PS-Simulink Converter  PhysicalDomain=network_engine_domain  SubClassName=ps_output  LeftPortType=input  RightPortType=output  PseudoPeriodic=off  Frequencies=[]  VectorFormat=1-D array  Unit=A  AffineConversion=off
  uu_afe : nesl_utility/PS-Simulink Converter  PhysicalDomain=network_engine_domain  SubClassName=ps_output  LeftPortType=input  RightPortType=output  PseudoPeriodic=off  Frequencies=[]  VectorFormat=1-D array  Unit=V  AffineConversion=off
  uv_afe : nesl_utility/PS-Simulink Converter  PhysicalDomain=network_engine_domain  SubClassName=ps_output  LeftPortType=input  RightPortType=output  PseudoPeriodic=off  Frequencies=[]  VectorFormat=1-D array  Unit=V  AffineConversion=off
  uw_afe : nesl_utility/PS-Simulink Converter  PhysicalDomain=network_engine_domain  SubClassName=ps_output  LeftPortType=input  RightPortType=output  PseudoPeriodic=off  Frequencies=[]  VectorFormat=1-D array  Unit=V  AffineConversion=off
  Uu : PMIOPort  Side=Left
  uu : PMIOPort  Port=2  Side=Right
  Uv : PMIOPort  Port=3  Side=Left
  uv : PMIOPort  Port=4  Side=Right
  Uw : PMIOPort  Port=5  Side=Left
  uw : PMIOPort  Port=6  Side=Right
  tag scope: i_im_uvw=global, u_im_uvw=global
  wires:
  Bus Creator/1 -> Selector1/1, Selector/1  "vi_data"
  Selector/1 -> [u_im_uvw]
  iv_inv/1 -> Bus Creator/5  "iv_inv"
  iu_inv/1 -> Bus Creator/4  "iu_inv"
  iw_inv/1 -> Bus Creator/6  "iw_inv"
  uu_afe/1 -> Bus Creator/1  "uu_afe"
  uv_afe/1 -> Bus Creator/2  "uv_afe"
  uw_afe/1 -> Bus Creator/3  "uw_afe"
  Selector1/1 -> [i_im_uvw]
  [i_im_uvw] -> i_im_uvw/u_im_uvw/1  "is_uvw"
  [u_im_uvw] -> i_im_uvw/u_im_uvw/2  "us_uvw"
  connections:
  Current Sensor1/LConn1 -- Uv/RConn1 -- Voltage Sensor1/LConn1
  Electrical Reference1/LConn1 -- Voltage Sensor/RConn2 -- Voltage Sensor2/RConn2 -- Voltage Sensor1/RConn2
  Voltage Sensor/RConn1 -- uu_afe/LConn1
  Current Sensor/RConn2 -- uu/RConn1
  Voltage Sensor1/RConn1 -- uv_afe/LConn1
  Voltage Sensor2/LConn1 -- Uw/RConn1 -- Current Sensor2/LConn1
  Current Sensor/LConn1 -- Uu/RConn1 -- Voltage Sensor/LConn1
  Current Sensor1/RConn2 -- uv/RConn1
  Voltage Sensor2/RConn1 -- uw_afe/LConn1
  iv_inv/LConn1 -- Current Sensor1/RConn1
  iu_inv/LConn1 -- Current Sensor/RConn1
  iw_inv/LConn1 -- Current Sensor2/RConn1
  Current Sensor2/RConn2 -- uw/RConn1

== system im_inv_sensorless_ctrl_model/inverter//ctrl/im_ctrl ==
  theta_m : Inport
  Bus Creator : BusCreator  Inputs=3
  Mux : Mux  Inputs=2
  Mux1 : Mux  Inputs=2
  Mux2 : Mux  Inputs=2
  abc2dq : Subsystem
  "abc2dq " : Subsystem
  acquisition : Subsystem
  dq2alphabeta : Subsystem
  im_control : Subsystem
  is_xy/umot : Scope  NumInputPorts=2
      settings: ActiveDisplayYMinimum=-2.1540901451739543  ActiveDisplayYMaximum=0.89534736379428759
  rotor_speed_observer : Subsystem
  u_ctrl_alphabeta : Outport  VectorParamsAs1DForOutWhenUnconnected=off
  tag scope: is_dq_pu_mod1=global, is_xy_pu_mod1=global, uctrl_out_alphabeta_mod1=global
  wires:
  Mux/1 -> [uctrl_out_alphabeta_mod1], u_ctrl_alphabeta/1
  Mux1/1 -> [is_xy_pu_mod1]
  im_control/1(usx) -> dq2alphabeta/1(x)
  im_control/2(usy) -> dq2alphabeta/2(y)
  dq2alphabeta/1(uctrl_alpha) -> Mux/1
  dq2alphabeta/2(uctrl_beta) -> Mux/2
  Mux2/1 -> [is_dq_pu_mod1]
  "abc2dq "/2(q) -> Mux2/2
  "abc2dq "/1(d) -> Mux2/1
  abc2dq/1(d) -> Mux1/1
  abc2dq/2(q) -> Mux1/2
  acquisition/2(iv) -> abc2dq/2(b), "abc2dq "/2(b)
  acquisition/1(iu) -> abc2dq/1(a), "abc2dq "/1(a)
  acquisition/3(iw) -> abc2dq/3(c), "abc2dq "/3(c)
  theta_m/1 -> "abc2dq "/4(wt)
  [theta_s_mod1] -> abc2dq/4(wt)
  im_control/3(theta_s) -> dq2alphabeta/3(theta_s)
  [is_xy_pu_mod1] -> is_xy/umot/1  "is_xy_pu_mod1"
  [ud_inv_mod1] -> Bus Creator/2  "ud"
  [um_ctrl_out_mod1] -> Bus Creator/1  "umot"
  [uq_inv_mod1] -> Bus Creator/3  "uq"
  Bus Creator/1 -> is_xy/umot/2

== system im_inv_sensorless_ctrl_model/inverter//ctrl/inverter ==
  uab : Inport
  Current Sensor : fl_lib/Electrical/Electrical Sensors/Current Sensor
  PS-Simulink Converter1 : nesl_utility/PS-Simulink Converter  PhysicalDomain=network_engine_domain  SubClassName=ps_output  LeftPortType=input  RightPortType=output  PseudoPeriodic=off  Frequencies=[]  VectorFormat=1-D array  Unit=A  AffineConversion=on
  PS-Simulink Converter4 : nesl_utility/PS-Simulink Converter  PhysicalDomain=network_engine_domain  SubClassName=ps_output  LeftPortType=input  RightPortType=output  PseudoPeriodic=off  Frequencies=[]  VectorFormat=1-D array  Unit=V  AffineConversion=on
  Transfer Fcn : TransferFcn  Denominator=[1e-2 1]
  Voltage Sensor : fl_lib/Electrical/Electrical Sensors/Voltage Sensor
  idc/udc : Scope  NumInputPorts=2
      settings: SampleTime=tc  ActiveDisplayYMinimum=-39.864272381805591  ActiveDisplayYMaximum=357.49537607008335
  inverter : Subsystem
  Udc(+) : PMIOPort  Side=Right
  Udc(-) : PMIOPort  Port=2  Side=Right
  us_u : PMIOPort  Port=3  Side=Left
  us_v : PMIOPort  Port=4  Side=Left
  us_w : PMIOPort  Port=5  Side=Left
  wires:
  uab/1 -> inverter/1(uab)
  Transfer Fcn/1 -> idc/udc/1  "idc_flt"
  PS-Simulink Converter1/1 -> Transfer Fcn/1  "idc"
  PS-Simulink Converter4/1 -> idc/udc/2  "udc"
  connections:
  PS-Simulink Converter1/LConn1 -- Current Sensor/RConn1
  Current Sensor/RConn2 -- inverter/RConn1 -- Voltage Sensor/LConn1
  Current Sensor/LConn1 -- Udc(+)/RConn1
  Udc(-)/RConn1 -- inverter/RConn2 -- Voltage Sensor/RConn2
  us_w/RConn1 -- inverter/LConn3
  us_v/RConn1 -- inverter/LConn2
  us_u/RConn1 -- inverter/LConn1
  PS-Simulink Converter4/LConn1 -- Voltage Sensor/RConn1

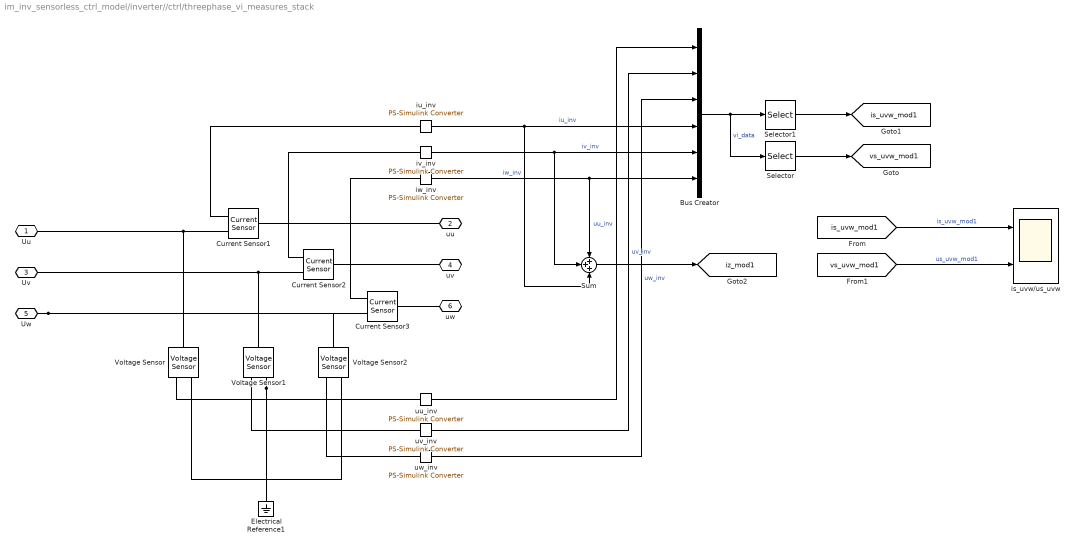
== system im_inv_sensorless_ctrl_model/inverter//ctrl/threephase_vi_measures_stack ==
  Bus Creator : BusCreator  Inputs=6
  Current Sensor1 : fl_lib/Electrical/Electrical Sensors/Current Sensor
  Current Sensor2 : fl_lib/Electrical/Electrical Sensors/Current Sensor
  Current Sensor3 : fl_lib/Electrical/Electrical Sensors/Current Sensor
  Electrical Reference1 : fl_lib/Electrical/Electrical Elements/Electrical Reference
  Selector : Selector  InputPortWidth=6  IndexOptions=Index vector (dialog)  Indices=[1 2 3]  OutputSizes=1
  Selector1 : Selector  InputPortWidth=6  IndexOptions=Index vector (dialog)  Indices=[4 5 6]  OutputSizes=1
  Sum : Sum  Inputs=+++
  Voltage Sensor : fl_lib/Electrical/Electrical Sensors/Voltage Sensor
  Voltage Sensor1 : fl_lib/Electrical/Electrical Sensors/Voltage Sensor
  Voltage Sensor2 : fl_lib/Electrical/Electrical Sensors/Voltage Sensor
  is_uvw/us_uvw : Scope  NumInputPorts=2
      settings: SampleTime=tc  ActiveDisplayYMinimum=-2616.6692677484148  ActiveDisplayYMaximum=2614.0144319252477
  iu_inv : nesl_utility/PS-Simulink Converter  PhysicalDomain=network_engine_domain  SubClassName=ps_output  LeftPortType=input  RightPortType=output  PseudoPeriodic=off  Frequencies=[]  VectorFormat=1-D array  Unit=A  AffineConversion=off
  iv_inv : nesl_utility/PS-Simulink Converter  PhysicalDomain=network_engine_domain  SubClassName=ps_output  LeftPortType=input  RightPortType=output  PseudoPeriodic=off  Frequencies=[]  VectorFormat=1-D array  Unit=A  AffineConversion=off
  iw_inv : nesl_utility/PS-Simulink Converter  PhysicalDomain=network_engine_domain  SubClassName=ps_output  LeftPortType=input  RightPortType=output  PseudoPeriodic=off  Frequencies=[]  VectorFormat=1-D array  Unit=A  AffineConversion=off
  uu_inv : nesl_utility/PS-Simulink Converter  PhysicalDomain=network_engine_domain  SubClassName=ps_output  LeftPortType=input  RightPortType=output  PseudoPeriodic=off  Frequencies=[]  VectorFormat=1-D array  Unit=V  AffineConversion=off
  uv_inv : nesl_utility/PS-Simulink Converter  PhysicalDomain=network_engine_domain  SubClassName=ps_output  LeftPortType=input  RightPortType=output  PseudoPeriodic=off  Frequencies=[]  VectorFormat=1-D array  Unit=V  AffineConversion=off
  uw_inv : nesl_utility/PS-Simulink Converter  PhysicalDomain=network_engine_domain  SubClassName=ps_output  LeftPortType=input  RightPortType=output  PseudoPeriodic=off  Frequencies=[]  VectorFormat=1-D array  Unit=V  AffineConversion=off
  Uu : PMIOPort  Side=Left
  uu : PMIOPort  Port=2  Side=Right
  Uv : PMIOPort  Port=3  Side=Left
  uv : PMIOPort  Port=4  Side=Right
  Uw : PMIOPort  Port=5  Side=Left
  uw : PMIOPort  Port=6  Side=Right
  tag scope: is_uvw_mod1=global, iz_mod1=global, vs_uvw_mod1=global
  wires:
  [vs_uvw_mod1] -> is_uvw/us_uvw/2  "us_uvw_mod1"
  [is_uvw_mod1] -> is_uvw/us_uvw/1  "is_uvw_mod1"
  uw_inv/1 -> Bus Creator/3  "uw_inv"
  uv_inv/1 -> Bus Creator/2  "uv_inv"
  uu_inv/1 -> Bus Creator/1  "uu_inv"
  iw_inv/1 -> Sum/1, Bus Creator/6  "iw_inv"
  iu_inv/1 -> Bus Creator/4, Sum/3  "iu_inv"
  iv_inv/1 -> Bus Creator/5, Sum/2  "iv_inv"
  Selector/1 -> [vs_uvw_mod1]
  Bus Creator/1 -> Selector/1, Selector1/1  "vi_data"
  Selector1/1 -> [is_uvw_mod1]
  Sum/1 -> [iz_mod1]
  connections:
  uw/RConn1 -- Current Sensor3/LConn1
  Voltage Sensor2/RConn1 -- uw_inv/LConn1
  Voltage Sensor/LConn1 -- Current Sensor1/RConn2 -- Uu/RConn1
  Uw/RConn1 -- Current Sensor3/RConn2 -- Voltage Sensor2/LConn1
  Voltage Sensor1/RConn1 -- uv_inv/LConn1
  Voltage Sensor/RConn1 -- uu_inv/LConn1
  Voltage Sensor1/RConn2 -- Voltage Sensor2/RConn2 -- Voltage Sensor/RConn2 -- Electrical Reference1/LConn1
  Voltage Sensor1/LConn1 -- Current Sensor2/RConn2 -- Uv/RConn1
  Current Sensor2/LConn1 -- uv/RConn1
  Current Sensor1/LConn1 -- uu/RConn1
  Current Sensor1/RConn1 -- iu_inv/LConn1
  Current Sensor2/RConn1 -- iv_inv/LConn1
  Current Sensor3/RConn1 -- iw_inv/LConn1

== system im_inv_sensorless_ctrl_model/induction motor/control performance evaluation/adc2dq_s_1 ==
  abc : Inport
  Bus Creator : BusCreator  Inputs=2
  abc2alphabeta : MATLAB Function  TreatAsAtomicUnit=on  SystemSampleTime=tc
  alphabeta2xieta : MATLAB Function  TreatAsAtomicUnit=on  SystemSampleTime=tc
  dq : Outport
  tag scope: psi_s_alpha_im=global, psi_s_beta_im=global
  wires:
  abc2alphabeta/1(alpha) -> [psi_s_alpha_im], alphabeta2xieta/1(alpha)  "alpha"
  abc2alphabeta/2(beta) -> [psi_s_beta_im], alphabeta2xieta/2(beta)  "beta"
  abc/1 -> abc2alphabeta/1(abc)
  [theta_s_mod1] -> alphabeta2xieta/3(theta)
  alphabeta2xieta/1(d) -> Bus Creator/1  "d"
  alphabeta2xieta/2(q) -> Bus Creator/2  "q"
  Bus Creator/1 -> dq/1

== system im_inv_sensorless_ctrl_model/induction motor/control performance evaluation/adc2dq_s_2 ==
  abc : Inport
  Bus Creator : BusCreator  Inputs=2
  abc2alphabeta : MATLAB Function  TreatAsAtomicUnit=on  SystemSampleTime=tc
  alphabeta2xieta : MATLAB Function  TreatAsAtomicUnit=on  SystemSampleTime=tc
  dq : Outport
  wires:
  Bus Creator/1 -> dq/1
  alphabeta2xieta/2(q) -> Bus Creator/2  "q"
  alphabeta2xieta/1(d) -> Bus Creator/1  "d"
  [theta_s_mod1] -> alphabeta2xieta/3(theta)
  abc/1 -> abc2alphabeta/1(abc)
  abc2alphabeta/2(beta) -> alphabeta2xieta/2(beta)  "beta"
  abc2alphabeta/1(alpha) -> alphabeta2xieta/1(alpha)  "alpha"

== system im_inv_sensorless_ctrl_model/induction motor/control performance evaluation/adc2dq_slip_1 ==
  abc : Inport
  Bus Creator : BusCreator  Inputs=2
  abc2alphabeta : MATLAB Function  TreatAsAtomicUnit=on  SystemSampleTime=tc
  alphabeta2xieta : MATLAB Function  TreatAsAtomicUnit=on  SystemSampleTime=tc
  dq : Outport
  wires:
  Bus Creator/1 -> dq/1
  alphabeta2xieta/2(q) -> Bus Creator/2  "q"
  alphabeta2xieta/1(d) -> Bus Creator/1  "d"
  [theta_slip_mod1] -> alphabeta2xieta/3(theta)
  abc/1 -> abc2alphabeta/1(abc)
  abc2alphabeta/2(beta) -> alphabeta2xieta/2(beta)  "beta"
  abc2alphabeta/1(alpha) -> alphabeta2xieta/1(alpha)  "alpha"

== system im_inv_sensorless_ctrl_model/induction motor/control performance evaluation/adc2dq_slip_2 ==
  abc : Inport
  Bus Creator : BusCreator  Inputs=2
  abc2alphabeta : MATLAB Function  TreatAsAtomicUnit=on  SystemSampleTime=tc
  alphabeta2xieta : MATLAB Function  TreatAsAtomicUnit=on  SystemSampleTime=tc
  dq : Outport
  wires:
  abc2alphabeta/1(alpha) -> alphabeta2xieta/1(alpha)  "alpha"
  abc2alphabeta/2(beta) -> alphabeta2xieta/2(beta)  "beta"
  abc/1 -> abc2alphabeta/1(abc)
  [theta_slip_mod1] -> alphabeta2xieta/3(theta)
  alphabeta2xieta/1(d) -> Bus Creator/1  "d"
  alphabeta2xieta/2(q) -> Bus Creator/2  "q"
  Bus Creator/1 -> dq/1
